simulink model "MotorExperiment"  (R2026b)
settings: Solver=ode4  StopTime=experimentCfg.Duration  FixedStep=experimentCfg.Step
PostLoadFcn:
  | addpath(fullfile(fileparts(fileparts(fileparts(fileparts(fileparts(fileparts(get_param(bdroot,'FileName'))))))),'docs','scripts'));initialize_motor_paths();initialize_motor_model(bdroot);
model workspace (MAT data in the model file):
  currentCfg.Ts = 0.0001
  currentCfg.BandwidthHz = 500
  currentCfg.Kpd = 3.14159265359
  currentCfg.Kpq = 3.76991118431
  currentCfg.Kid = 1570.79632679
  currentCfg.Kiq = 1570.79632679
  currentCfg.Kaw = 1000
  deadtimeCfg.DeadTime = 2e-06
  deadtimeCfg.DeviceDrop = 0
  deadtimeCfg.CurrentBlend = 0.1
  deadtimeCfg.ModelEnable = 0
  deadtimeCfg.CompensationEnable = 0
  deadtimeCfg.CompensationScale = 1
  deadtimeCfg.SwitchingStep = 1e-07
  experimentCfg.Step = 5e-06
  experimentCfg.LogTs = 0.0001
  experimentCfg.Duration = 1.5
  experimentCfg.Mode = 2
  experimentCfg.UseInverter = 1
  experimentCfg.UseTiming = 1
  experimentCfg.UseMechanical = 1
  experimentCfg.ImposedElectricalSpeed = 0
  experimentCfg.IdReference = 0
  experimentCfg.IqReference = 2
  experimentCfg.IqInitial = 0
  experimentCfg.SpeedReference = 40
  experimentCfg.SpeedInitial = 0
  experimentCfg.PositionReference = 1
  experimentCfg.PositionInitial = 0
  experimentCfg.CommandTime = 0.05
  experimentCfg.LoadTorque = 0.1
  experimentCfg.LoadTime = 0.35
  experimentCfg.Enable = 1
  experimentCfg.Reset = 0
  feedforwardCfg.Enable = 0
  feedforwardCfg.ParameterScale = 1
  fixtureCfg.Ts = 0.0001
  fixtureCfg.Duration = 1.5
  fixtureCfg.SolverStep = 5e-06
  fixtureCfg.Inputs = [0; 0]
  inverterCfg.Vdc = 48
  inverterCfg.MinDuty = 0.02
  inverterCfg.PwmTs = 0.0001
  inverterCfg.LinearLimit = 26.6043004043
  motionCfg.Ts = 0.001
  motionCfg.NaturalFrequency = 20
  motionCfg.Damping = 0.9
  motionCfg.Kt = 0.21
  motionCfg.Kp = 0.0852380952381
  motionCfg.Ki = 0.952380952381
  motionCfg.Kaw = 20
  motionCfg.PositionKp = 8
  motionCfg.SpeedLimit = 80
  motionCfg.AccelerationLimit = 200
  motionCfg.CurrentLimit = 8
  pmsmCfg.Rs = 0.5
  pmsmCfg.Ld = 0.001
  pmsmCfg.Lq = 0.0012
  pmsmCfg.Flux = 0.035
  pmsmCfg.PolePairs = 4
  pmsmCfg.J = 0.0005
  pmsmCfg.B = 0.0001
  pmsmCfg.Id0 = 0
  pmsmCfg.Iq0 = 0
  pmsmCfg.Speed0 = 0
  pmsmCfg.Position0 = 0
  testStim.time = []
  testStim.signals.values = [0; 0]
  testStim.signals.dimensions = 1
  timingCfg.Ts = 0.0001
  timingCfg.FeedbackTicks = 1
  timingCfg.ActuationTicks = 1
libraries: ClarkePark x11, Inverter x3, CurrentControl x2, PMSMPlant x2, ControlTiming x2, MotionControl x2, Deadtime x2, DQFeedforward x1
settings Model: Creator=24322  LastModifiedBy=24322

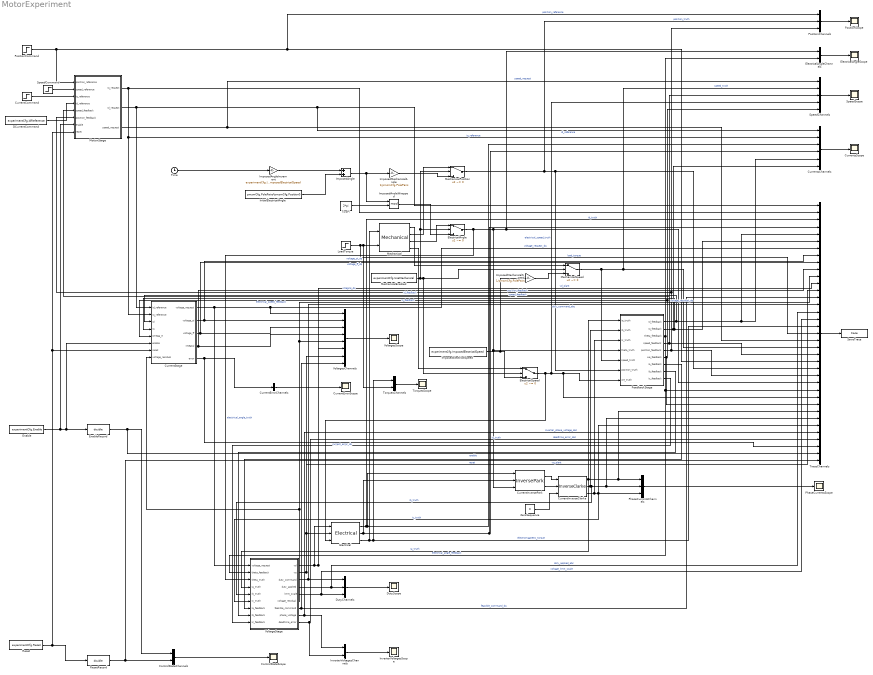
== system MotorExperiment ==
  ControlStateChannels : Mux  Inputs=2
  ControlStateScope : Scope
      settings: Title=ControlState  YLabel=1
  CurrentCommand : Step  Time=experimentCfg.CommandTime  InitialValue=experimentCfg.IqInitial  FinalValue=experimentCfg.IqReference  SampleTime=currentCfg.Ts
  CurrentErrorChannels : Mux  Inputs=1
  CurrentErrorScope : Scope
      settings: Title=CurrentError  YLabel=A
  CurrentInverseClarke : ClarkePark/InverseClarke  SystemSampleTime=-1  VariantActivationTime=update diagram  EmptyChoice=off  PassThrough=off  PassThroughVariantControl=(default)  EmptyChoiceVariantControl=(default)  AllowFlexibleInterface=on  Latency=0  AutoFrameSizeCalculation=off
  CurrentInversePark : ClarkePark/InversePark  SystemSampleTime=-1  VariantActivationTime=update diagram  EmptyChoice=off  PassThrough=off  PassThroughVariantControl=(default)  EmptyChoiceVariantControl=(default)  AllowFlexibleInterface=on  Latency=0  AutoFrameSizeCalculation=off
  CurrentStage : Subsystem
  CurrentsChannels : Mux  Inputs=6
  CurrentsScope : Scope
      settings: Title=Currents  YLabel=A
  DCurrentCommand : Constant  Value=experimentCfg.IdReference
  DutyChannels : Mux  Inputs=3
  DutyScope : Scope
      settings: Title=Duty  YLabel=1
  Electrical : PMSMPlant/Electrical  SystemSampleTime=-1  VariantActivationTime=update diagram  EmptyChoice=off  PassThrough=off  PassThroughVariantControl=(default)  EmptyChoiceVariantControl=(default)  AllowFlexibleInterface=on  Latency=0  AutoFrameSizeCalculation=off
  ElectricalAngle : Switch  Criteria=u2 ~= 0  SaturateOnIntegerOverflow=off  InputSameDT=off
  ElectricalAngleChannels : Mux  Inputs=2
  ElectricalAngleScope : Scope
      settings: Title=ElectricalAngle  YLabel=rad
  ElectricalSpeed : Switch  Criteria=u2 ~= 0  SaturateOnIntegerOverflow=off  InputSameDT=off
  Enable : Constant  Value=experimentCfg.Enable  OutDataTypeStr=boolean
  EnableRecord : DataTypeConversion  OutDataTypeStr=double  SaturateOnIntegerOverflow=off  RndMeth=Floor
  FeedbackStage : Subsystem
  ImposedAngle : Sum
  ImposedAngleIncrement : Gain  Gain=experimentCfg.ImposedElectricalSpeed
  ImposedAngleWrapped : Math  Operator=mod
  ImposedElectricalSpeed : Constant  Value=experimentCfg.ImposedElectricalSpeed
  ImposedMechanicalAngle : Gain  Gain=1/pmsmCfg.PolePairs
  ImposedMechanicalSpeed : Gain  Gain=1/pmsmCfg.PolePairs
  InitialElectricalAngle : Constant  Value=pmsmCfg.PolePairs*pmsmCfg.Position0
  InverterVoltagesChannels : Mux  Inputs=2
  InverterVoltagesScope : Scope
      settings: Title=InverterVoltages  YLabel=V
  LoadTorque : Step  Time=experimentCfg.LoadTime  FinalValue=experimentCfg.LoadTorque  SampleTime=currentCfg.Ts
  Mechanical : PMSMPlant/Mechanical  SystemSampleTime=-1  VariantActivationTime=update diagram  EmptyChoice=off  PassThrough=off  PassThroughVariantControl=(default)  EmptyChoiceVariantControl=(default)  AllowFlexibleInterface=on  Latency=0  AutoFrameSizeCalculation=off
  MechanicalEnabled : Constant  Value=experimentCfg.UseMechanical
  MechanicalPosition : Switch  Criteria=u2 ~= 0  SaturateOnIntegerOverflow=off  InputSameDT=off
  MechanicalSpeed : Switch  Criteria=u2 ~= 0  SaturateOnIntegerOverflow=off  InputSameDT=off
  MotionStage : Subsystem
  PhaseCurrentsChannels : Mux  Inputs=3
  PhaseCurrentsScope : Scope
      settings: Title=PhaseCurrents  YLabel=A
  PositionChannels : Mux  Inputs=3
  PositionCommand : Step  Time=experimentCfg.CommandTime  InitialValue=experimentCfg.PositionInitial  FinalValue=experimentCfg.PositionReference  SampleTime=motionCfg.Ts
  PositionScope : Scope
      settings: Title=Position  ActiveDisplayYMinimum=-0.74998749999999992  ActiveDisplayYMaximum=6.7498875  YLabel=rad
  Reset : Constant  Value=experimentCfg.Reset  OutDataTypeStr=boolean
  ResetRecord : DataTypeConversion  OutDataTypeStr=double  SaturateOnIntegerOverflow=off  RndMeth=Floor
  SaveTrace : ToWorkspace  VariableName=trace  SaveFormat=Structure With Time  SampleTime=experimentCfg.LogTs
  SpeedChannels : Mux  Inputs=5
  SpeedCommand : Step  Time=experimentCfg.CommandTime  InitialValue=experimentCfg.SpeedInitial  FinalValue=experimentCfg.SpeedReference  SampleTime=motionCfg.Ts
  SpeedScope : Scope
      settings: Title=Speed  YLabel=rad/s
  Time : Clock
  TorquesChannels : Mux  Inputs=2
  TorquesScope : Scope
      settings: Title=Torques  YLabel=N*m
  TraceChannels : Mux  Inputs=37
  TwoPi : Constant  Value=2*pi
  VoltageStage : Subsystem
  VoltagesChannels : Mux  Inputs=8
  VoltagesScope : Scope
      settings: Title=Voltages  YLabel=V
  ZeroSequence : Constant  Value=0
  wires:
  ControlStateChannels/1 -> ControlStateScope/1
  CurrentErrorChannels/1 -> CurrentErrorScope/1
  InverterVoltagesChannels/1 -> InverterVoltagesScope/1
  PhaseCurrentsChannels/1 -> PhaseCurrentsScope/1
  ElectricalAngleChannels/1 -> ElectricalAngleScope/1
  PositionChannels/1 -> PositionScope/1
  SpeedChannels/1 -> SpeedScope/1
  TorquesChannels/1 -> TorquesScope/1
  DutyChannels/1 -> DutyScope/1
  VoltagesChannels/1 -> VoltagesScope/1
  CurrentsChannels/1 -> CurrentsScope/1
  ResetRecord/1 -> TraceChannels/37, ControlStateChannels/2  "reset"
  EnableRecord/1 -> TraceChannels/36, ControlStateChannels/1  "enable"
  CurrentStage/5(error) -> TraceChannels/35, CurrentErrorChannels/1  "current_error_dq"
  VoltageStage/9(deadtime_error) -> TraceChannels/34, InverterVoltagesChannels/2  "deadtime_error_abc"
  VoltageStage/8(phase_voltage) -> TraceChannels/33, InverterVoltagesChannels/1  "inverter_phase_voltage_abc"
  MotionStage/3(speed_request) -> TraceChannels/20, SpeedChannels/1  "speed_request"
  VoltageStage/5(limit_scale) -> TraceChannels/17, DutyChannels/3  "voltage_limit_scale"
  VoltageStage/4(duty_applied) -> TraceChannels/16, DutyChannels/2  "duty_applied_abc"
  VoltageStage/3(duty_command) -> TraceChannels/15, DutyChannels/1  "duty_command_abc"
  VoltageStage/7(feasible_command) -> TraceChannels/14, VoltagesChannels/8  "feasible_command_dq"
  CurrentStage/4(integral) -> TraceChannels/10, VoltagesChannels/4  "integral_dq"
  CurrentStage/3(voltage_ff) -> TraceChannels/9, VoltagesChannels/3  "voltage_ff_dq"
  CurrentStage/2(voltage_pi) -> TraceChannels/8, VoltagesChannels/2  "voltage_pi_dq"
  TraceChannels/1 -> SaveTrace/1
  FeedbackStage/9(ic_feedback) -> VoltageStage/9(ic_feedback)
  FeedbackStage/8(ib_feedback) -> VoltageStage/8(ib_feedback)
  FeedbackStage/7(ia_feedback) -> VoltageStage/7(ia_feedback)
  FeedbackStage/3(theta_feedback) -> VoltageStage/2(theta_feedback), TraceChannels/27, ElectricalAngleChannels/2  "electrical_angle_feedback"
  CurrentStage/1(voltage_request) -> TraceChannels/7, VoltagesChannels/1, VoltageStage/1(voltage_request)  "voltage_request_dq"
  VoltageStage/6(voltage_residual) -> TraceChannels/11, VoltagesChannels/5, CurrentStage/8(voltage_residual)  "voltage_residual_dq"
  FeedbackStage/6(we_feedback) -> SpeedChannels/5, CurrentStage/5(omega_e), TraceChannels/29  "electrical_speed_feedback"
  FeedbackStage/2(iq_feedback) -> CurrentStage/4(iq), TraceChannels/6, CurrentsChannels/6  "iq_feedback"
  FeedbackStage/1(id_feedback) -> CurrentsChannels/5, TraceChannels/5, CurrentStage/3(id)  "id_feedback"
  MotionStage/1(iq_request) -> CurrentsChannels/2, CurrentStage/2(iq_reference), TraceChannels/2  "iq_reference"
  MotionStage/2(id_request) -> TraceChannels/1, CurrentsChannels/1, CurrentStage/1(id_reference)  "id_reference"
  Reset/1 -> MotionStage/8(reset), CurrentStage/7(reset), ResetRecord/1
  Enable/1 -> CurrentStage/6(enable), EnableRecord/1, MotionStage/7(enable)
  FeedbackStage/5(position_feedback) -> MotionStage/6(position_feedback), PositionChannels/3, TraceChannels/25  "position_feedback"
  FeedbackStage/4(speed_feedback) -> TraceChannels/22, MotionStage/5(speed_feedback), SpeedChannels/3  "speed_feedback"
  DCurrentCommand/1 -> MotionStage/4(id_reference)
  CurrentCommand/1 -> MotionStage/3(iq_reference)
  SpeedCommand/1 -> MotionStage/2(speed_reference)
  PositionCommand/1 -> TraceChannels/23, PositionChannels/1, MotionStage/1(position_reference)  "position_reference"
  MechanicalPosition/1 -> FeedbackStage/6(position_truth), TraceChannels/24, PositionChannels/2  "position_truth"
  MechanicalSpeed/1 -> TraceChannels/21, SpeedChannels/2, FeedbackStage/5(speed_truth)  "speed_truth"
  CurrentInverseClarke/3 -> TraceChannels/32, PhaseCurrentsChannels/3, VoltageStage/6(ic_truth), FeedbackStage/3(ic_truth)  "ic_truth"
  CurrentInverseClarke/2 -> TraceChannels/31, PhaseCurrentsChannels/2, VoltageStage/5(ib_truth), FeedbackStage/2(ib_truth)  "ib_truth"
  CurrentInverseClarke/1 -> PhaseCurrentsChannels/1, TraceChannels/30, FeedbackStage/1(ia_truth), VoltageStage/4(ia_truth)  "ia_truth"
  ZeroSequence/1 -> CurrentInverseClarke/3
  CurrentInversePark/2 -> CurrentInverseClarke/2
  CurrentInversePark/1 -> CurrentInverseClarke/1
  ElectricalAngle/1 -> CurrentInversePark/3, FeedbackStage/4(theta_truth), ElectricalAngleChannels/1, TraceChannels/26, VoltageStage/3(theta_truth)  "electrical_angle_truth"
  Electrical/2 -> TraceChannels/4, CurrentsChannels/4, CurrentInversePark/2  "iq_truth"
  Electrical/1 -> CurrentsChannels/3, CurrentInversePark/1, TraceChannels/3  "id_truth"
  Mechanical/4 -> ElectricalSpeed/1
  ImposedAngleWrapped/1 -> ElectricalAngle/3
  Mechanical/3 -> ElectricalAngle/1
  ImposedMechanicalAngle/1 -> MechanicalPosition/3
  Mechanical/2 -> MechanicalPosition/1
  ImposedMechanicalSpeed/1 -> MechanicalSpeed/3
  MechanicalEnabled/1 -> MechanicalSpeed/2, ElectricalSpeed/2, MechanicalPosition/2, ElectricalAngle/2
  Mechanical/1 -> MechanicalSpeed/1
  TwoPi/1 -> ImposedAngleWrapped/2
  ImposedAngle/1 -> ImposedMechanicalAngle/1, ImposedAngleWrapped/1
  InitialElectricalAngle/1 -> ImposedAngle/2
  ImposedAngleIncrement/1 -> ImposedAngle/1
  Time/1 -> ImposedAngleIncrement/1
  ImposedElectricalSpeed/1 -> ImposedMechanicalSpeed/1, ElectricalSpeed/3
  VoltageStage/2(vq) -> Electrical/2, VoltagesChannels/7, TraceChannels/13  "vq_plant"
  VoltageStage/1(vd) -> VoltagesChannels/6, TraceChannels/12, Electrical/1  "vd_plant"
  ElectricalSpeed/1 -> FeedbackStage/7(we_truth), TraceChannels/28, SpeedChannels/4, Electrical/3  "electrical_speed_truth"
  LoadTorque/1 -> TorquesChannels/2, Mechanical/2, TraceChannels/19  "load_torque"
  Electrical/3 -> TorquesChannels/1, TraceChannels/18, Mechanical/1  "electromagnetic_torque"

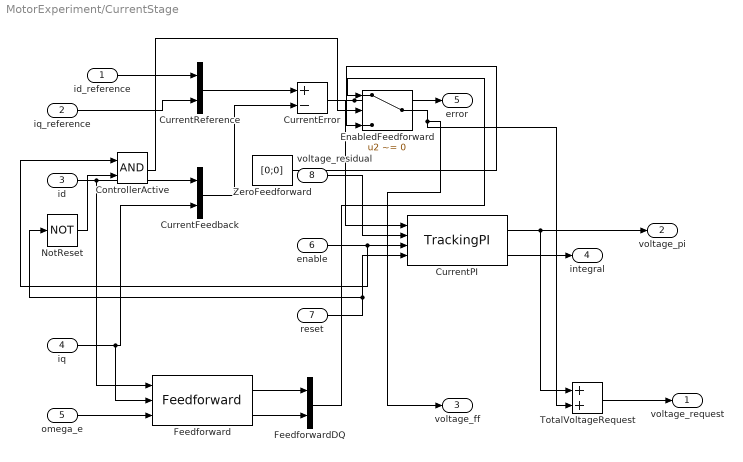
== system MotorExperiment/CurrentStage ==
  id_reference : Inport
  iq_reference : Inport  Port=2
  id : Inport  Port=3
  iq : Inport  Port=4
  omega_e : Inport  Port=5
  enable : Inport  Port=6
  reset : Inport  Port=7
  voltage_residual : Inport  Port=8
  ControllerActive : Logic  AllPortsSameDT=off  OutDataTypeStr=boolean
  CurrentError : Sum  Inputs=+-
  CurrentFeedback : Mux  Inputs=2
  CurrentPI : CurrentControl/TrackingPI  SystemSampleTime=-1  VariantActivationTime=update diagram  EmptyChoice=off  PassThrough=off  PassThroughVariantControl=(default)  EmptyChoiceVariantControl=(default)  AllowFlexibleInterface=on  Latency=0  AutoFrameSizeCalculation=off
  CurrentReference : Mux  Inputs=2
  EnabledFeedforward : Switch  Criteria=u2 ~= 0  SaturateOnIntegerOverflow=off  InputSameDT=off
  Feedforward : DQFeedforward/Feedforward  SystemSampleTime=-1  VariantActivationTime=update diagram  EmptyChoice=off  PassThrough=off  PassThroughVariantControl=(default)  EmptyChoiceVariantControl=(default)  AllowFlexibleInterface=on  Latency=0  AutoFrameSizeCalculation=off
  FeedforwardDQ : Mux  Inputs=2
  NotReset : Logic  Operator=NOT  AllPortsSameDT=off  OutDataTypeStr=boolean
  TotalVoltageRequest : Sum
  ZeroFeedforward : Constant  Value=[0;0]
  voltage_request : Outport
  voltage_pi : Outport  Port=2
  voltage_ff : Outport  Port=3
  integral : Outport  Port=4
  error : Outport  Port=5
  wires:
  CurrentPI/2 -> integral/1
  TotalVoltageRequest/1 -> voltage_request/1
  CurrentPI/1 -> TotalVoltageRequest/1, voltage_pi/1
  Feedforward/2 -> FeedforwardDQ/2
  Feedforward/1 -> FeedforwardDQ/1
  omega_e/1 -> Feedforward/3
  reset/1 -> CurrentPI/4, NotReset/1
  enable/1 -> ControllerActive/1, CurrentPI/3
  voltage_residual/1 -> CurrentPI/2
  CurrentError/1 -> error/1, CurrentPI/1
  CurrentFeedback/1 -> CurrentError/2
  CurrentReference/1 -> CurrentError/1
  iq/1 -> CurrentFeedback/2, Feedforward/2
  id/1 -> CurrentFeedback/1, Feedforward/1
  iq_reference/1 -> CurrentReference/2
  id_reference/1 -> CurrentReference/1
  EnabledFeedforward/1 -> voltage_ff/1, TotalVoltageRequest/2
  ZeroFeedforward/1 -> EnabledFeedforward/3
  ControllerActive/1 -> EnabledFeedforward/2
  NotReset/1 -> ControllerActive/2
  FeedforwardDQ/1 -> EnabledFeedforward/1

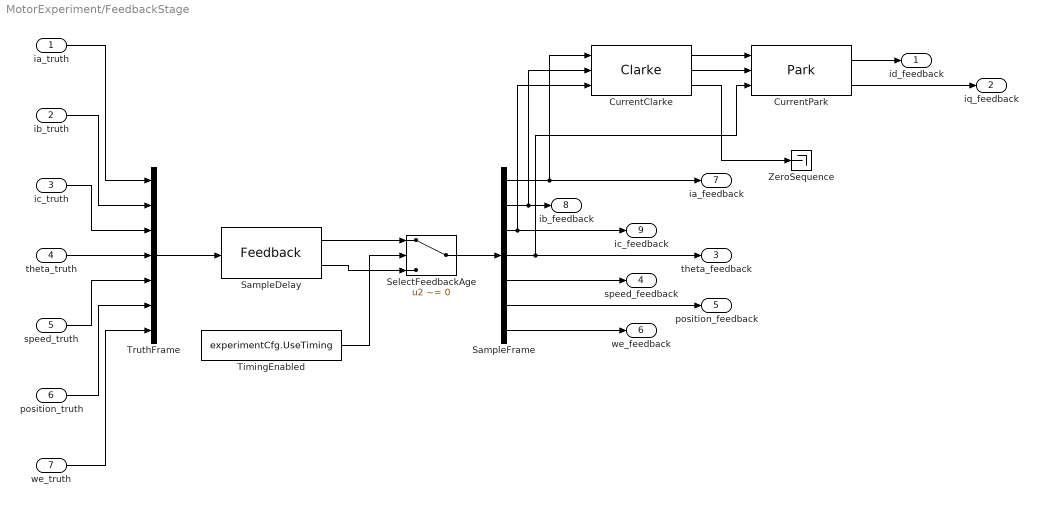
== system MotorExperiment/FeedbackStage ==
  ia_truth : Inport
  ib_truth : Inport  Port=2
  ic_truth : Inport  Port=3
  theta_truth : Inport  Port=4
  speed_truth : Inport  Port=5
  position_truth : Inport  Port=6
  we_truth : Inport  Port=7
  CurrentClarke : ClarkePark/Clarke  SystemSampleTime=-1  VariantActivationTime=update diagram  EmptyChoice=off  PassThrough=off  PassThroughVariantControl=(default)  EmptyChoiceVariantControl=(default)  AllowFlexibleInterface=on  Latency=0  AutoFrameSizeCalculation=off
  CurrentPark : ClarkePark/Park  SystemSampleTime=-1  VariantActivationTime=update diagram  EmptyChoice=off  PassThrough=off  PassThroughVariantControl=(default)  EmptyChoiceVariantControl=(default)  AllowFlexibleInterface=on  Latency=0  AutoFrameSizeCalculation=off
  SampleDelay : ControlTiming/Feedback  SystemSampleTime=-1  VariantActivationTime=update diagram  EmptyChoice=off  PassThrough=off  PassThroughVariantControl=(default)  EmptyChoiceVariantControl=(default)  AllowFlexibleInterface=on  Latency=0  AutoFrameSizeCalculation=off
  SampleFrame : Demux  Outputs=7
  SelectFeedbackAge : Switch  Criteria=u2 ~= 0  SaturateOnIntegerOverflow=off  InputSameDT=off
  TimingEnabled : Constant  Value=experimentCfg.UseTiming
  TruthFrame : Mux  Inputs=7
  ZeroSequence : Terminator
  id_feedback : Outport
  iq_feedback : Outport  Port=2
  theta_feedback : Outport  Port=3
  speed_feedback : Outport  Port=4
  position_feedback : Outport  Port=5
  we_feedback : Outport  Port=6
  ia_feedback : Outport  Port=7
  ib_feedback : Outport  Port=8
  ic_feedback : Outport  Port=9
  wires:
  SampleFrame/7 -> we_feedback/1
  SampleFrame/6 -> position_feedback/1
  SampleFrame/5 -> speed_feedback/1
  CurrentPark/2 -> iq_feedback/1
  CurrentPark/1 -> id_feedback/1
  CurrentClarke/3 -> ZeroSequence/1
  SampleFrame/4 -> CurrentPark/3, theta_feedback/1
  CurrentClarke/2 -> CurrentPark/2
  CurrentClarke/1 -> CurrentPark/1
  SampleFrame/3 -> CurrentClarke/3, ic_feedback/1
  SampleFrame/2 -> CurrentClarke/2, ib_feedback/1
  SampleFrame/1 -> CurrentClarke/1, ia_feedback/1
  SelectFeedbackAge/1 -> SampleFrame/1
  SampleDelay/2 -> SelectFeedbackAge/3
  TimingEnabled/1 -> SelectFeedbackAge/2
  SampleDelay/1 -> SelectFeedbackAge/1
  TruthFrame/1 -> SampleDelay/1
  we_truth/1 -> TruthFrame/7
  position_truth/1 -> TruthFrame/6
  speed_truth/1 -> TruthFrame/5
  theta_truth/1 -> TruthFrame/4
  ic_truth/1 -> TruthFrame/3
  ib_truth/1 -> TruthFrame/2
  ia_truth/1 -> TruthFrame/1

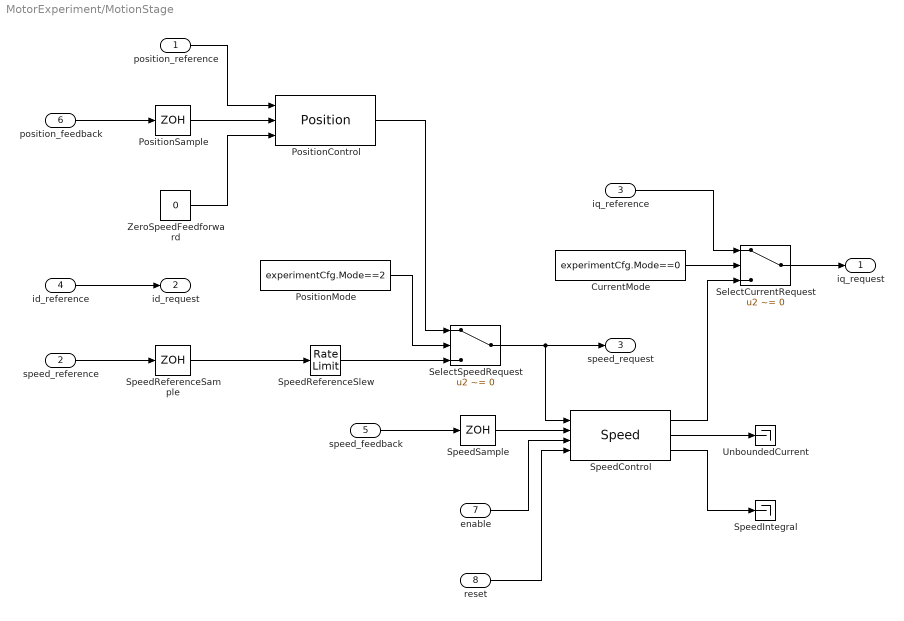
== system MotorExperiment/MotionStage ==
  position_reference : Inport
  speed_reference : Inport  Port=2
  iq_reference : Inport  Port=3
  id_reference : Inport  Port=4
  speed_feedback : Inport  Port=5
  position_feedback : Inport  Port=6
  enable : Inport  Port=7
  reset : Inport  Port=8
  CurrentMode : Constant  Value=experimentCfg.Mode==0
  PositionControl : MotionControl/Position  SystemSampleTime=-1  VariantActivationTime=update diagram  EmptyChoice=off  PassThrough=off  PassThroughVariantControl=(default)  EmptyChoiceVariantControl=(default)  AllowFlexibleInterface=on  Latency=0  AutoFrameSizeCalculation=off
  PositionMode : Constant  Value=experimentCfg.Mode==2
  PositionSample : ZeroOrderHold  SampleTime=motionCfg.Ts
  SelectCurrentRequest : Switch  Criteria=u2 ~= 0  SaturateOnIntegerOverflow=off  InputSameDT=off
  SelectSpeedRequest : Switch  Criteria=u2 ~= 0  SaturateOnIntegerOverflow=off  InputSameDT=off
  SpeedControl : MotionControl/Speed  SystemSampleTime=-1  VariantActivationTime=update diagram  EmptyChoice=off  PassThrough=off  PassThroughVariantControl=(default)  EmptyChoiceVariantControl=(default)  AllowFlexibleInterface=on  Latency=0  AutoFrameSizeCalculation=off
  SpeedIntegral : Terminator
  SpeedReferenceSample : ZeroOrderHold  SampleTime=motionCfg.Ts
  SpeedReferenceSlew : RateLimiter  RisingSlewLimit=motionCfg.AccelerationLimit  FallingSlewLimit=-motionCfg.AccelerationLimit  SampleTimeMode=inherited
  SpeedSample : ZeroOrderHold  SampleTime=motionCfg.Ts
  UnboundedCurrent : Terminator
  ZeroSpeedFeedforward : Constant  Value=0
  iq_request : Outport
  id_request : Outport  Port=2
  speed_request : Outport  Port=3
  wires:
  id_reference/1 -> id_request/1
  SelectCurrentRequest/1 -> iq_request/1
  SpeedControl/3 -> SpeedIntegral/1
  SpeedControl/2 -> UnboundedCurrent/1
  SpeedControl/1 -> SelectCurrentRequest/3
  CurrentMode/1 -> SelectCurrentRequest/2
  iq_reference/1 -> SelectCurrentRequest/1
  reset/1 -> SpeedControl/4
  enable/1 -> SpeedControl/3
  SpeedSample/1 -> SpeedControl/2
  SelectSpeedRequest/1 -> SpeedControl/1, speed_request/1
  SpeedReferenceSlew/1 -> SelectSpeedRequest/3
  PositionMode/1 -> SelectSpeedRequest/2
  PositionControl/1 -> SelectSpeedRequest/1
  SpeedReferenceSample/1 -> SpeedReferenceSlew/1
  speed_reference/1 -> SpeedReferenceSample/1
  ZeroSpeedFeedforward/1 -> PositionControl/3
  PositionSample/1 -> PositionControl/2
  position_reference/1 -> PositionControl/1
  speed_feedback/1 -> SpeedSample/1
  position_feedback/1 -> PositionSample/1

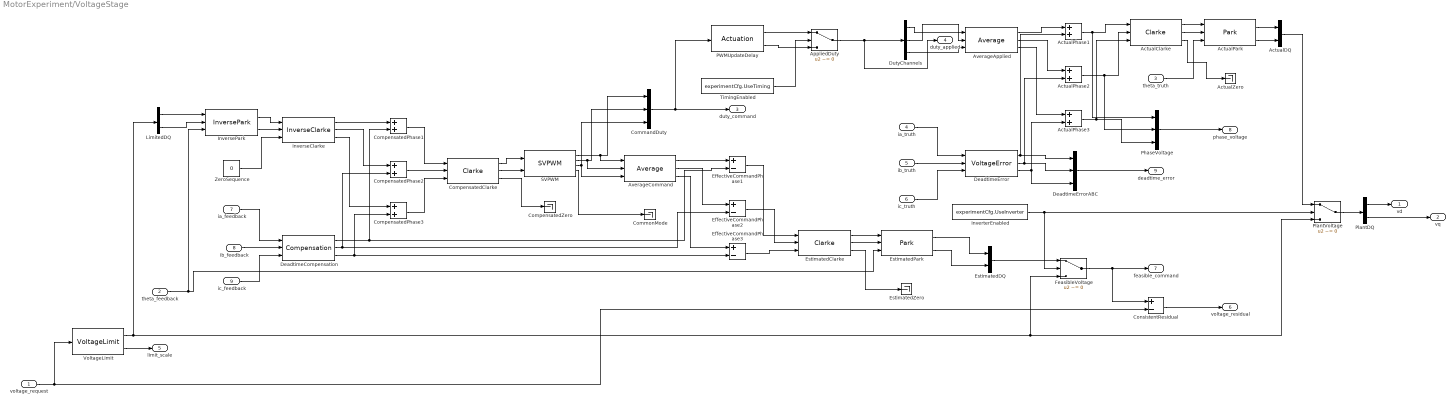
== system MotorExperiment/VoltageStage ==
  voltage_request : Inport
  theta_feedback : Inport  Port=2
  theta_truth : Inport  Port=3
  ia_truth : Inport  Port=4
  ib_truth : Inport  Port=5
  ic_truth : Inport  Port=6
  ia_feedback : Inport  Port=7
  ib_feedback : Inport  Port=8
  ic_feedback : Inport  Port=9
  ActualClarke : ClarkePark/Clarke  SystemSampleTime=-1  VariantActivationTime=update diagram  EmptyChoice=off  PassThrough=off  PassThroughVariantControl=(default)  EmptyChoiceVariantControl=(default)  AllowFlexibleInterface=on  Latency=0  AutoFrameSizeCalculation=off
  ActualDQ : Mux  Inputs=2
  ActualPark : ClarkePark/Park  SystemSampleTime=-1  VariantActivationTime=update diagram  EmptyChoice=off  PassThrough=off  PassThroughVariantControl=(default)  EmptyChoiceVariantControl=(default)  AllowFlexibleInterface=on  Latency=0  AutoFrameSizeCalculation=off
  ActualPhase1 : Sum
  ActualPhase2 : Sum
  ActualPhase3 : Sum
  ActualZero : Terminator
  AppliedDuty : Switch  Criteria=u2 ~= 0  SaturateOnIntegerOverflow=off  InputSameDT=off
  AverageApplied : Inverter/Average  SystemSampleTime=-1  VariantActivationTime=update diagram  EmptyChoice=off  PassThrough=off  PassThroughVariantControl=(default)  EmptyChoiceVariantControl=(default)  AllowFlexibleInterface=on  Latency=0  AutoFrameSizeCalculation=off
  AverageCommand : Inverter/Average  SystemSampleTime=-1  VariantActivationTime=update diagram  EmptyChoice=off  PassThrough=off  PassThroughVariantControl=(default)  EmptyChoiceVariantControl=(default)  AllowFlexibleInterface=on  Latency=0  AutoFrameSizeCalculation=off
  CommandDuty : Mux  Inputs=3
  CommonMode : Terminator
  CompensatedClarke : ClarkePark/Clarke  SystemSampleTime=-1  VariantActivationTime=update diagram  EmptyChoice=off  PassThrough=off  PassThroughVariantControl=(default)  EmptyChoiceVariantControl=(default)  AllowFlexibleInterface=on  Latency=0  AutoFrameSizeCalculation=off
  CompensatedPhase1 : Sum
  CompensatedPhase2 : Sum
  CompensatedPhase3 : Sum
  CompensatedZero : Terminator
  ConsistentResidual : Sum  Inputs=+-
  DeadtimeCompensation : Deadtime/Compensation  SystemSampleTime=-1  VariantActivationTime=update diagram  EmptyChoice=off  PassThrough=off  PassThroughVariantControl=(default)  EmptyChoiceVariantControl=(default)  AllowFlexibleInterface=on  Latency=0  AutoFrameSizeCalculation=off
  DeadtimeError : Deadtime/VoltageError  SystemSampleTime=-1  VariantActivationTime=update diagram  EmptyChoice=off  PassThrough=off  PassThroughVariantControl=(default)  EmptyChoiceVariantControl=(default)  AllowFlexibleInterface=on  Latency=0  AutoFrameSizeCalculation=off
  DeadtimeErrorABC : Mux  Inputs=3
  DutyChannels : Demux  Outputs=3
  EffectiveCommandPhase1 : Sum  Inputs=+-
  EffectiveCommandPhase2 : Sum  Inputs=+-
  EffectiveCommandPhase3 : Sum  Inputs=+-
  EstimatedClarke : ClarkePark/Clarke  SystemSampleTime=-1  VariantActivationTime=update diagram  EmptyChoice=off  PassThrough=off  PassThroughVariantControl=(default)  EmptyChoiceVariantControl=(default)  AllowFlexibleInterface=on  Latency=0  AutoFrameSizeCalculation=off
  EstimatedDQ : Mux  Inputs=2
  EstimatedPark : ClarkePark/Park  SystemSampleTime=-1  VariantActivationTime=update diagram  EmptyChoice=off  PassThrough=off  PassThroughVariantControl=(default)  EmptyChoiceVariantControl=(default)  AllowFlexibleInterface=on  Latency=0  AutoFrameSizeCalculation=off
  EstimatedZero : Terminator
  FeasibleVoltage : Switch  Criteria=u2 ~= 0  SaturateOnIntegerOverflow=off  InputSameDT=off
  InverseClarke : ClarkePark/InverseClarke  SystemSampleTime=-1  VariantActivationTime=update diagram  EmptyChoice=off  PassThrough=off  PassThroughVariantControl=(default)  EmptyChoiceVariantControl=(default)  AllowFlexibleInterface=on  Latency=0  AutoFrameSizeCalculation=off
  InversePark : ClarkePark/InversePark  SystemSampleTime=-1  VariantActivationTime=update diagram  EmptyChoice=off  PassThrough=off  PassThroughVariantControl=(default)  EmptyChoiceVariantControl=(default)  AllowFlexibleInterface=on  Latency=0  AutoFrameSizeCalculation=off
  InverterEnabled : Constant  Value=experimentCfg.UseInverter
  LimitedDQ : Demux  Outputs=2
  PWMUpdateDelay : ControlTiming/Actuation  SystemSampleTime=-1  VariantActivationTime=update diagram  EmptyChoice=off  PassThrough=off  PassThroughVariantControl=(default)  EmptyChoiceVariantControl=(default)  AllowFlexibleInterface=on  Latency=0  AutoFrameSizeCalculation=off
  PhaseVoltage : Mux  Inputs=3
  PlantDQ : Demux  Outputs=2
  PlantVoltage : Switch  Criteria=u2 ~= 0  SaturateOnIntegerOverflow=off  InputSameDT=off
  SVPWM : Inverter/SVPWM  SystemSampleTime=-1  VariantActivationTime=update diagram  EmptyChoice=off  PassThrough=off  PassThroughVariantControl=(default)  EmptyChoiceVariantControl=(default)  AllowFlexibleInterface=on  Latency=0  AutoFrameSizeCalculation=off
  TimingEnabled : Constant  Value=experimentCfg.UseTiming
  VoltageLimit : CurrentControl/VoltageLimit  SystemSampleTime=-1  VariantActivationTime=update diagram  EmptyChoice=off  PassThrough=off  PassThroughVariantControl=(default)  EmptyChoiceVariantControl=(default)  AllowFlexibleInterface=on  Latency=0  AutoFrameSizeCalculation=off
  ZeroSequence : Constant  Value=0
  vd : Outport
  vq : Outport  Port=2
  duty_command : Outport  Port=3
  duty_applied : Outport  Port=4
  limit_scale : Outport  Port=5
  voltage_residual : Outport  Port=6
  feasible_command : Outport  Port=7
  phase_voltage : Outport  Port=8
  deadtime_error : Outport  Port=9
  wires:
  EffectiveCommandPhase3/1 -> EstimatedClarke/3
  AverageCommand/3 -> EffectiveCommandPhase3/1
  ActualPhase3/1 -> ActualClarke/3, PhaseVoltage/3
  DeadtimeError/3 -> ActualPhase3/2, DeadtimeErrorABC/3
  AverageApplied/3 -> ActualPhase3/1
  DutyChannels/3 -> AverageApplied/3
  SVPWM/3 -> CommandDuty/3, AverageCommand/3
  CompensatedPhase3/1 -> CompensatedClarke/3
  DeadtimeCompensation/3 -> CompensatedPhase3/2, EffectiveCommandPhase3/2
  InverseClarke/3 -> CompensatedPhase3/1
  ic_truth/1 -> DeadtimeError/3
  ic_feedback/1 -> DeadtimeCompensation/3
  EffectiveCommandPhase2/1 -> EstimatedClarke/2
  AverageCommand/2 -> EffectiveCommandPhase2/1
  ActualPhase2/1 -> ActualClarke/2, PhaseVoltage/2
  DeadtimeError/2 -> ActualPhase2/2, DeadtimeErrorABC/2
  AverageApplied/2 -> ActualPhase2/1
  DutyChannels/2 -> AverageApplied/2
  SVPWM/2 -> CommandDuty/2, AverageCommand/2
  CompensatedPhase2/1 -> CompensatedClarke/2
  DeadtimeCompensation/2 -> CompensatedPhase2/2, EffectiveCommandPhase2/2
  InverseClarke/2 -> CompensatedPhase2/1
  ib_truth/1 -> DeadtimeError/2
  ib_feedback/1 -> DeadtimeCompensation/2
  EffectiveCommandPhase1/1 -> EstimatedClarke/1
  AverageCommand/1 -> EffectiveCommandPhase1/1
  ActualPhase1/1 -> ActualClarke/1, PhaseVoltage/1
  DeadtimeError/1 -> ActualPhase1/2, DeadtimeErrorABC/1
  AverageApplied/1 -> ActualPhase1/1
  DutyChannels/1 -> AverageApplied/1
  SVPWM/1 -> CommandDuty/1, AverageCommand/1
  CompensatedPhase1/1 -> CompensatedClarke/1
  DeadtimeCompensation/1 -> CompensatedPhase1/2, EffectiveCommandPhase1/2
  InverseClarke/1 -> CompensatedPhase1/1
  ia_truth/1 -> DeadtimeError/1
  ia_feedback/1 -> DeadtimeCompensation/1
  DeadtimeErrorABC/1 -> deadtime_error/1
  PhaseVoltage/1 -> phase_voltage/1
  ConsistentResidual/1 -> voltage_residual/1
  VoltageLimit/2 -> limit_scale/1
  PlantDQ/2 -> vq/1
  PlantDQ/1 -> vd/1
  PlantVoltage/1 -> PlantDQ/1
  FeasibleVoltage/1 -> ConsistentResidual/1, feasible_command/1
  EstimatedDQ/1 -> FeasibleVoltage/1
  InverterEnabled/1 -> PlantVoltage/2, FeasibleVoltage/2
  ActualDQ/1 -> PlantVoltage/1
  EstimatedPark/2 -> EstimatedDQ/2
  EstimatedPark/1 -> EstimatedDQ/1
  ActualPark/2 -> ActualDQ/2
  ActualPark/1 -> ActualDQ/1
  EstimatedClarke/3 -> EstimatedZero/1
  EstimatedClarke/2 -> EstimatedPark/2
  EstimatedClarke/1 -> EstimatedPark/1
  ActualClarke/3 -> ActualZero/1
  theta_truth/1 -> ActualPark/3
  ActualClarke/2 -> ActualPark/2
  ActualClarke/1 -> ActualPark/1
  AppliedDuty/1 -> DutyChannels/1, duty_applied/1
  PWMUpdateDelay/2 -> AppliedDuty/3
  TimingEnabled/1 -> AppliedDuty/2
  PWMUpdateDelay/1 -> AppliedDuty/1
  CommandDuty/1 -> PWMUpdateDelay/1, duty_command/1
  SVPWM/4 -> CommonMode/1
  CompensatedClarke/3 -> CompensatedZero/1
  CompensatedClarke/2 -> SVPWM/2
  CompensatedClarke/1 -> SVPWM/1
  ZeroSequence/1 -> InverseClarke/3
  InversePark/2 -> InverseClarke/2
  InversePark/1 -> InverseClarke/1
  theta_feedback/1 -> InversePark/3, EstimatedPark/3
  LimitedDQ/2 -> InversePark/2
  LimitedDQ/1 -> InversePark/1
  VoltageLimit/1 -> PlantVoltage/3, FeasibleVoltage/3, LimitedDQ/1
  voltage_request/1 -> ConsistentResidual/2, VoltageLimit/1
